simulink model "Transmission_Line_Model1"  (R2024a)
settings: Solver=FixedStepAuto  StartTime=0.0  StopTime=0.25  FixedStep=4.62962962962963e-05  RelTol=1e-3
libraries: spsRMSLib x4, spsThreePhaseSeriesRLCBranchLib x2, spsPower3phInstantaneousLib x2, spsThreePhaseVIMeasurementLib x2, spsThreePhaseSeriesRLCLoadLib x1, spsThreePhaseFaultLib x1, spsThreePhaseSourceLib x1, sps_lib x1
settings Model: Creator=ludwi  LastModifiedBy=ludwi

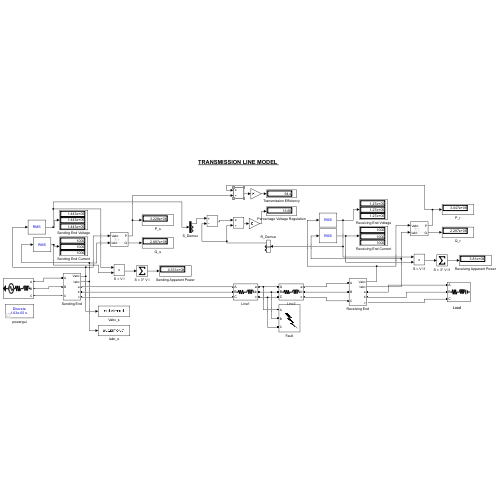
[thumbnail: Simulink's stored preview of the top-level diagram]
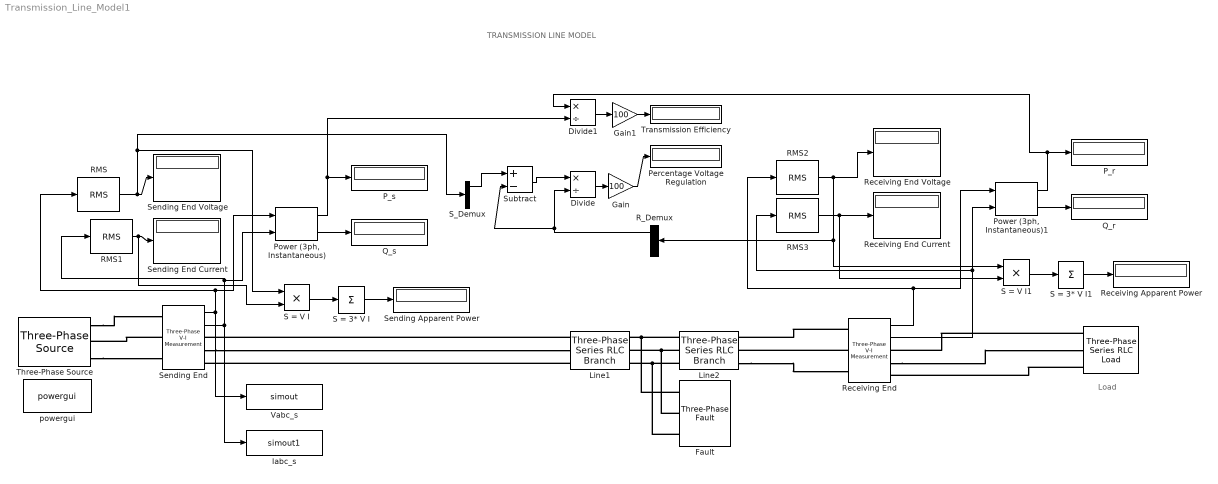
== system Transmission_Line_Model1 ==
  note: Load
  note: TRANSMISSION LINE MODEL
  " " : spsThreePhaseSeriesRLCLoadLib/Three-Phase Series RLC Load  LConnTagsString=A|B|C  Configuration=Y (grounded)  NominalVoltage=220e3  Vabc=[1e3 1e3 1e3]  Vabcp=[1e3 1e3 1e3]  NominalFrequency=60  UnbalancedPower=off  ActivePower=304.8e6  InductivePower=228.8e6  CapacitivePower=0  Pabc=[10e3 9e3 11e3]  QLabc=[100 90 110]  QCabc=[100 90 110]  Pabcp=[10e3 9e3 11e3]  QLabcp=[100 90 110]  QCabcp=[100 90 110]  Measurements=None  LoadType=constant Z
  Divide : Product  Inputs=*/
  Divide1 : Product  Inputs=*/
  Fault : spsThreePhaseFaultLib/Three-Phase Fault  InitialStates=0  FaultA=on  FaultB=off  FaultC=off  GroundFault=off  SwitchTimes=[100]  External=off  SwitchStatus=NaN  FaultResistance=29.17  GroundResistance=29.17  SnubberResistance=1e6  SnubberCapacitance=inf  Measurements=None
  Gain : Gain  Gain=100
  Gain1 : Gain  Gain=100
  Iabc_s : ToWorkspace  VariableName=simout1  SaveFormat=Timeseries  SampleTime=-1
  Line1 : spsThreePhaseSeriesRLCBranchLib/Three-Phase Series RLC Branch  LConnTagsString=A|B|C  RConnTagsString=A|B|C  BranchType=RL  Resistance=2.38837  Inductance=0.021118  Capacitance=1e-6  Measurements=None
  Line2 : spsThreePhaseSeriesRLCBranchLib/Three-Phase Series RLC Branch  LConnTagsString=A|B|C  RConnTagsString=A|B|C  BranchType=RL  Resistance=3.61163  Inductance=0.031934  Capacitance=1e-6  Measurements=None
  P_r : Display
  P_s : Display
  Percentage Voltage Regulation : Display
  "Power (3ph, Instantaneous)" : spsPower3phInstantaneousLib/Power (3ph, Instantaneous)
  "Power (3ph, Instantaneous)1" : spsPower3phInstantaneousLib/Power (3ph, Instantaneous)
  Q_r : Display
  Q_s : Display
  RMS : spsRMSLib/RMS  TrueRMS=on  Freq=60  RMSInit=0  Ts=0
  RMS1 : spsRMSLib/RMS  TrueRMS=on  Freq=60  RMSInit=120  Ts=0
  RMS2 : spsRMSLib/RMS  TrueRMS=on  Freq=60  RMSInit=0  Ts=0
  RMS3 : spsRMSLib/RMS  TrueRMS=on  Freq=60  RMSInit=120  Ts=0
  R_Demux : Demux  Outputs=3
      settings: DisplayOption=none
  Receiving Apparent Power : Display
  Receiving End : spsThreePhaseVIMeasurementLib/Three-Phase V-I Measurement  VoltageMeasurement=phase-to-ground  SetLabelV=off  LabelV=Vabc  Vpu=off  VpuLL=off  CurrentMeasurement=yes  SetLabelI=off  LabelI=Iabc  Ipu=off  Pbase=100e6  Vbase=500e3  OutputType=Complex  PhasorSimulation=off  PSBequivalent=0
  Receiving End Current : Display
  Receiving End Voltage : Display
  S = 3* V I : Sum  Inputs=+
  S = 3* V I1 : Sum  Inputs=+
  S = V I : Product
  S = V I1 : Product
  S_Demux : Demux  Outputs=3
  Sending Apparent Power : Display
  Sending End : spsThreePhaseVIMeasurementLib/Three-Phase V-I Measurement  VoltageMeasurement=phase-to-ground  SetLabelV=off  LabelV=Vabc  Vpu=off  VpuLL=off  CurrentMeasurement=yes  SetLabelI=off  LabelI=Iabc  Ipu=off  Pbase=100e6  Vbase=500e3  OutputType=Complex  PhasorSimulation=off  PSBequivalent=0
  Sending End Current : Display
  Sending End Voltage : Display
  Subtract : Sum  Inputs=+-
  Three-Phase Source : spsThreePhaseSourceLib/Three-Phase Source  InternalConnection=Yg  VoltagePhases=off  Voltage=263.1e3  PhaseAngle=0  Voltage_phases=[25e3 25e3 25e3]/sqrt(3)  PhaseAngles_phases=[0 -120 +120]  Frequency=60  NonIdealSource=on  SpecifyImpedance=off  Resistance=1  Inductance=26.526e-3  ShortCircuitLevel=100e6  BaseVoltage=25e3  XRratio=7  BusType=swing  Pref=10e3  Qref=0  Prefabc=[10e3, 10e3, 10e3]  Qrefabc=[0, 0, 0]  Qmin=-inf  Qmax=inf
  Transmission Efficiency : Display
  Vabc_s : ToWorkspace  VariableName=simout  SaveFormat=Timeseries  SampleTime=-1
  powergui : sps_lib/powergui  Priority=1  SimulationMode=Discrete  SampleTime=4.62962962962963e-05  frequency=60  Iterations=50  frequencyindice=60  Pbase=100e6  ErrMax=1e-4  UnitsV=kV  UnitsW=MW  buscounter=0  FunctionMessages=off  echomessages=off  EnableUseOfTLC=off  CurrentSourceSwitches=off  DisableSnubberDevices=off  DisableRonSwitches=off  DisableVfSwitches=off  DisplayEquations=off  AutomaticDiscreteSolvers=off  SolverType=Tustin/Backward Euler (TBE)  Interpol=off  ExternalGateDelay=off  methode=off  Ts=100  x0status=blocks  SPID=on  SwTol=0  HookPort=off  NonlinearTolerance=1e-4  nMaxIteration=100  ContinueOnMaxIteration=off  RestoreLinks=warning  ResistiveCurrentMeasurement=off  Frange=[0:2:500]  Ylog=off  Xlog=on  ShowGrid=off  save=off  variable=ZData  structure=0  ZoomFFT=off  StartTime=0.0  cycles=1  DisplayStyle=1  fundamental=60  FreqAxis=off  MaxFrequency=1000  frequencyindicesteady=1  RmsSteady=1  display=off
  wires:
  Sending End/1 -> RMS/1, "Power (3ph, Instantaneous)"/1, Vabc_s/1
  RMS1/1 -> S = V I/2, Sending End Current/1
  Sending End/2 -> "Power (3ph, Instantaneous)"/2, RMS1/1, Iabc_s/1
  "Power (3ph, Instantaneous)"/1 -> Divide1/2, P_s/1
  "Power (3ph, Instantaneous)"/2 -> Q_s/1
  S = V I/1 -> S = 3* V I/1
  S = 3* V I/1 -> Sending Apparent Power/1
  "Power (3ph, Instantaneous)1"/1 -> P_r/1, Divide1/1
  "Power (3ph, Instantaneous)1"/2 -> Q_r/1
  S = V I1/1 -> S = 3* V I1/1
  RMS2/1 -> S = V I1/1, R_Demux/1, Receiving End Voltage/1
  S = 3* V I1/1 -> Receiving Apparent Power/1
  RMS3/1 -> S = V I1/2, Receiving End Current/1
  Receiving End/1 -> "Power (3ph, Instantaneous)1"/1, RMS2/1
  Receiving End/2 -> "Power (3ph, Instantaneous)1"/2, RMS3/1
  RMS/1 -> S_Demux/1, S = V I/1, Sending End Voltage/1
  Subtract/1 -> Divide/1
  Divide/1 -> Gain/1
  S_Demux/1 -> Subtract/1
  Gain/1 -> Percentage Voltage Regulation/1
  R_Demux/1 -> Divide/2, Subtract/2
  Divide1/1 -> Gain1/1
  Gain1/1 -> Transmission Efficiency/1
  connections:
  Three-Phase Source/RConn1 -- Sending End/LConn1
  Sending End/LConn2 -- Three-Phase Source/RConn2
  Three-Phase Source/RConn3 -- Sending End/LConn3
  Line1/LConn1 -- Sending End/RConn1
  Sending End/RConn2 -- Line1/LConn2
  Line1/LConn3 -- Sending End/RConn3
  " "/LConn1 -- Receiving End/RConn1
  Receiving End/RConn2 -- " "/LConn2
  " "/LConn3 -- Receiving End/RConn3
  Line2/LConn1 -- Fault/LConn1 -- Line1/RConn1
  Line2/LConn2 -- Line1/RConn2 -- Fault/LConn2
  Line2/LConn3 -- Line1/RConn3 -- Fault/LConn3
  Receiving End/LConn1 -- Line2/RConn1
  Receiving End/LConn2 -- Line2/RConn2
  Line2/RConn3 -- Receiving End/LConn3
